simulink model "RobustFormationControl_IntegerModel_under_Dis"  (R2023a)
settings: Solver=ode3  StartTime=0.0  StopTime=30  FixedStep=0.0001  RelTol=1e-3
InitFcn:
  | % % Parameters for the fractional order NTFSMC:
  | % Sliding Surface " Sx, Sy, and Sz ":
  | %------------------------
  | % 10
  | % 10
  | cx = 2*[4 4 4];
  | cxx = 1*[0.01 0.01 0.01];
  | 
  | cx1 = cx(1);
  | cy1 = cx(2);
  | cz1 = cx(3);
  | 
  | cx2 = cxx(1);
  | cy2 = cxx(2);
  | cz2 = cxx(3);
  | 
  | alpha1 = [0.6 0.6 0.6];
  | alpha2 = [0.1 0.1 0.1];
  | 
  | gammaX = [3 3 3];
  | gx  = gammaX(1);
  | gy = gammaX(2);
  | gz = gammaX(3);
  | 
  | p = 10;
  | q = 10;
  | 
  | % Sliding Surface " S_Phi , S_Theta, and  S_Psi":
  | %------------------------
  | cP = 2*[4 4 4];
  | cPP = 1*[0.01 0.01 0.01 0.01];
  | 
  | cPhi1 = cP(1);
  | cTheta1 = cP(2);
  | cPsi1 = cP(3);
  | 
  | cPhi2 = cPP(1);
  | cTheta2 = cPP(2);
  | cPsi2 = cPP(3);
  | gammaP = [3 3 3];
  | 
  | %=========================
  | %=========================
  | SigmaX = 1*[0.01 0.01 0.01];
  | SigmaXX =1*[1 1 1];
  | 
  | Sigma1X = SigmaX(1);
  | Sigma1Y = SigmaX(2);
  | Sigma1Z = SigmaX(3);
  | %-----
  | Sigma2X = SigmaXX(1);
  | Sigma2Y = SigmaXX(2);
  | Sigma2Z = SigmaXX(3);
  | 
  | 
  | SigmaP = 1*[0.01 0.01 0.01];
  | SigmaPP =1*[1 1 1];
  | 
  | Sigma1Phi   = SigmaP(1);
  | Sigma1Theta = SigmaP(2);
  | ... (+80 lines)
values from neighbouring files (symbols this model uses):
  a1 = (Iyy - Izz)/Ixx    (= -0.812397034596)    [init_quadrotor_params.m]
  a2 = (Izz - Ixx)/Iyy    (= 0.812397034596)    [init_quadrotor_params.m]
  a3 = (Ixx - Iyy)/Izz    (= 0)    [init_quadrotor_params.m]
  a4 = - Ktx/m    (= -0.00114547325103)    [init_quadrotor_params.m]
  a5 = - Kty/m    (= -0.00114547325103)    [init_quadrotor_params.m]
  a6 = - Ktz/m    (= -0.00130740740741)    [init_quadrotor_params.m]
  b = 2.980e-5    (= 2.98e-05)    [init_quadrotor_params.m]
  b1 = - Jr/Ixx    (= -0.00584534596376)    [init_quadrotor_params.m]
  b2 = Jr/Iyy    (= 0.00584534596376)    [init_quadrotor_params.m]
  b3 = - Kfz/Izz    (= -0.0721963413248)    [init_quadrotor_params.m]
  b4 = 1/m    (= 2.05761316872)    [init_quadrotor_params.m]
  b5 = 1/m    (= 2.05761316872)    [init_quadrotor_params.m]
  b6 = 1/m    (= 2.05761316872)    [init_quadrotor_params.m]
  c1 = - Kfx/Ixx    (= -0.114641680395)    [init_quadrotor_params.m]
  c2 = - Kfy/Iyy    (= -0.114641680395)    [init_quadrotor_params.m]
  c3 = 1/Izz    (= 113.62345188)    [init_quadrotor_params.m]
  d = 1.12e-06    [init_quadrotor_params.m]
  d1 = L/Ixx    (= 46.334431631)    [init_quadrotor_params.m]
  d2 = L/Iyy    (= 46.334431631)    [init_quadrotor_params.m]
  g = 9.81    [init_quadrotor_params.m]
  Ixx = 4.856e-3    (= 0.004856)    [init_quadrotor_params.m]
  Iyy = 4.856e-3    (= 0.004856)    [init_quadrotor_params.m]
  Izz = 8.801e-3    (= 0.008801)    [init_quadrotor_params.m]
  Jr = 2.8385e-5    (= 2.8385e-05)    [init_quadrotor_params.m]
  Kfx = 5.567e-4    (= 0.0005567)    [init_quadrotor_params.m]
  Kfy = 5.567e-4    (= 0.0005567)    [init_quadrotor_params.m]
  Kfz = 6.354e-4    (= 0.0006354)    [init_quadrotor_params.m]
  Ktx = 5.5670e-4    (= 0.0005567)    [init_quadrotor_params.m]
  Kty = 5.5670e-4    (= 0.0005567)    [init_quadrotor_params.m]
  Ktz = 6.3540e-4    (= 0.0006354)    [init_quadrotor_params.m]
  L = 0.225    [init_quadrotor_params.m]
  m = 0.486    [init_quadrotor_params.m]
libraries: fod x120, eeStairGenerator x5
(part 3 of 9)

== system RobustFormationControl_IntegerModel_under_Dis/Integer Leader and four followers/Follower 3 System/Follower 2 Quadrotor Model/Quadrotor Dynamic System ==
  U1 : Inport
  U2 : Inport  Port=2
  U3 : Inport  Port=3
  U4 : Inport  Port=4
  Ux : Inport  Port=5
  Uy : Inport  Port=6
  Omega : Inport  Port=7
  Rotational System : Subsystem
  Translational System : Subsystem
  x = x7 : Outport  VectorParamsAs1DForOutWhenUnconnected=off
  y = x9 : Outport  Port=2  VectorParamsAs1DForOutWhenUnconnected=off
  z = x11 : Outport  Port=3  VectorParamsAs1DForOutWhenUnconnected=off
  Phi : Outport  Port=4  VectorParamsAs1DForOutWhenUnconnected=off
  Theta : Outport  Port=5  VectorParamsAs1DForOutWhenUnconnected=off
  Psi : Outport  Port=6  VectorParamsAs1DForOutWhenUnconnected=off
  x2 : Outport  Port=7  VectorParamsAs1DForOutWhenUnconnected=off
  x4 : Outport  Port=8  VectorParamsAs1DForOutWhenUnconnected=off
  x6 : Outport  Port=9  VectorParamsAs1DForOutWhenUnconnected=off
  xdot = x8 : Outport  Port=10  VectorParamsAs1DForOutWhenUnconnected=off
  ydot = x10 : Outport  Port=11  VectorParamsAs1DForOutWhenUnconnected=off
  zdot = x12 : Outport  Port=12  VectorParamsAs1DForOutWhenUnconnected=off
  wires:
  Rotational System/6(x6) -> x6/1
  Rotational System/5(x4) -> x4/1
  Rotational System/4(x2) -> x2/1
  Translational System/6(zdot or x12) -> zdot = x12/1
  Translational System/5(ydot or x10) -> ydot = x10/1
  Translational System/4(xdot or x8) -> xdot = x8/1
  Uy/1 -> Translational System/3(Uy)
  Ux/1 -> Translational System/2(Ux)
  Translational System/1(x or x7) -> x = x7/1  "X"
  Translational System/2(y or x9) -> y = x9/1  "Y"
  U1/1 -> Translational System/1(U1)
  Omega/1 -> Rotational System/4(Omega)
  Translational System/3(z or x11) -> z = x11/1  "Z"
  Rotational System/3(Psi or x5) -> Psi/1  "Psi"
  U3/1 -> Rotational System/2(U3)
  U2/1 -> Rotational System/1(U2)
  U4/1 -> Rotational System/3(U4)
  Rotational System/1(Phi or x1) -> Phi/1, Translational System/4(x1)  "Phi"
  Rotational System/2(Theta or x3) -> Theta/1, Translational System/5(x3)  "Theta"

== system RobustFormationControl_IntegerModel_under_Dis/Integer Leader and four followers/Follower 4 System/Desired Values/Helical Trajectry ==
  t : Inport
  Gain2 : Gain  Gain=0.2
  Step1 : Step  Time=0  SampleTime=0
  Trigonometric Function : Trigonometry
  Trigonometric Function1 : Trigonometry  Operator=cos
  xd : Outport  VectorParamsAs1DForOutWhenUnconnected=off
  yd : Outport  Port=2  VectorParamsAs1DForOutWhenUnconnected=off
  zd : Outport  Port=3  VectorParamsAs1DForOutWhenUnconnected=off
  Psi_d : Outport  Port=4  VectorParamsAs1DForOutWhenUnconnected=off
  wires:
  t/1 -> Trigonometric Function1/1, Trigonometric Function/1, Gain2/1
  Gain2/1 -> zd/1
  Step1/1 -> Psi_d/1
  Trigonometric Function1/1 -> xd/1
  Trigonometric Function/1 -> yd/1

== system RobustFormationControl_IntegerModel_under_Dis/Integer Leader and four followers/Follower 4 System/Desired Values/Helical Trajectry1 ==
  t : Inport
  Gain : Gain  Gain=dis
  Gain1 : Gain  Gain=2*pi/15
  Gain2 : Gain  Gain=1/15
  Gain3 : Gain  Gain=2*pi/15
  Scope : Scope
  Step : Step  Time=0  After=0  SampleTime=0.03
  Step1 : Step  Time=0  SampleTime=0
  Step2 : Step  Time=5  After=0.5  SampleTime=0.03
  Step3 : Step  Time=10  After=0.5  SampleTime=0.03
  Sum : Sum  Inputs=++-
  Sum1 : Sum  Inputs=|++
  Trigonometric Function : Trigonometry  Operator=cos
  Trigonometric Function1 : Trigonometry
  xd : Outport  VectorParamsAs1DForOutWhenUnconnected=off
  yd : Outport  Port=2  VectorParamsAs1DForOutWhenUnconnected=off
  zd : Outport  Port=3  VectorParamsAs1DForOutWhenUnconnected=off
  Psi_d : Outport  Port=4  VectorParamsAs1DForOutWhenUnconnected=off
  wires:
  t/1 -> Gain1/1, Gain3/1, Gain2/1
  Gain2/1 -> zd/1
  Step1/1 -> Psi_d/1
  Trigonometric Function1/1 -> yd/1
  Step/1 -> Sum/1
  Sum/1 -> Gain/1, Scope/1
  Step2/1 -> Sum/2
  Step3/1 -> Sum/3
  Sum1/1 -> xd/1
  Trigonometric Function/1 -> Sum1/2
  Gain/1 -> Sum1/1
  Gain1/1 -> Trigonometric Function/1
  Gain3/1 -> Trigonometric Function1/1

== system RobustFormationControl_IntegerModel_under_Dis/Integer Leader and four followers/Follower 4 System/Desired Values/Step Inputs Trajectry ==
  Step : Step  Time=0  After=3  SampleTime=0
  Step1 : Step  Time=0  After=5  SampleTime=0
  Step2 : Step  Time=0  SampleTime=0
  Step3 : Step  Time=0  After=2  SampleTime=0
  xd : Outport  VectorParamsAs1DForOutWhenUnconnected=off
  yd : Outport  Port=2  VectorParamsAs1DForOutWhenUnconnected=off
  zd : Outport  Port=3  VectorParamsAs1DForOutWhenUnconnected=off
  Psi_d : Outport  Port=4  VectorParamsAs1DForOutWhenUnconnected=off
  wires:
  Step2/1 -> xd/1
  Step3/1 -> yd/1
  Step/1 -> zd/1
  Step1/1 -> Psi_d/1

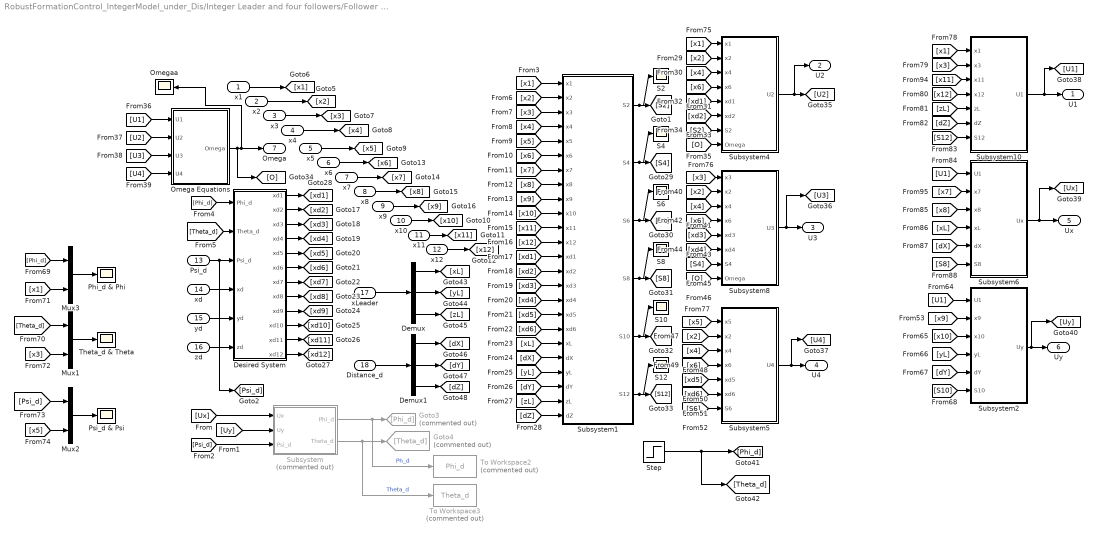
== system RobustFormationControl_IntegerModel_under_Dis/Integer Leader and four followers/Follower 4 System/Follower 2 Quadrotor Model/Control Module1 ==
  x1 : Inport
  x2 : Inport  Port=2
  x3 : Inport  Port=3
  x4 : Inport  Port=4
  x5 : Inport  Port=5
  x6 : Inport  Port=6
  x7 : Inport  Port=7
  x8 : Inport  Port=8
  x9 : Inport  Port=9
  x10 : Inport  Port=10
  x11 : Inport  Port=11
  x12 : Inport  Port=12
  Psi_d : Inport  Port=13
  " xd" : Inport  Port=14
  yd : Inport  Port=15
  " zd" : Inport  Port=16
  xLeader : Inport  Port=17
  Distance_d : Inport  Port=18
  " Phi_d & Phi" : Scope
  " Theta_d & Theta" : Scope
  Demux : Demux  Outputs=3
  Demux1 : Demux  Outputs=3
  Desired System : Subsystem
  Goto3 : Goto  Commented=on  GotoTag=Phi_d
  Goto4 : Goto  Commented=on  GotoTag=Theta_d
  Mux1 : Mux  Inputs=2
  Mux2 : Mux  Inputs=2
  Mux3 : Mux  Inputs=2
  Omega Equations : Subsystem
  Omegaa : Scope
  Psi_d & Psi : Scope
  S{4,6,8,10,12} (5 alike) : Scope
  "S2 " : Scope
  Step : Step  Time=0  After=0.001  SampleTime=0
  Subsystem : Subsystem  Commented=on
  Subsystem1 : Subsystem
  Subsystem10 : Subsystem
  Subsystem2 : Subsystem
  Subsystem4 : Subsystem
  Subsystem5 : Subsystem
  Subsystem6 : Subsystem
  Subsystem8 : Subsystem
  To Workspace2 : ToWorkspace  Commented=on  VariableName=Phi_d  SampleTime=-1
  To Workspace3 : ToWorkspace  Commented=on  VariableName=Theta_d  SampleTime=-1
  U1 : Outport  VectorParamsAs1DForOutWhenUnconnected=off
  U2 : Outport  Port=2  VectorParamsAs1DForOutWhenUnconnected=off
  U3 : Outport  Port=3  VectorParamsAs1DForOutWhenUnconnected=off
  U4 : Outport  Port=4  VectorParamsAs1DForOutWhenUnconnected=off
  Ux : Outport  Port=5  VectorParamsAs1DForOutWhenUnconnected=off
  Uy : Outport  Port=6  VectorParamsAs1DForOutWhenUnconnected=off
  Omega : Outport  Port=7  VectorParamsAs1DForOutWhenUnconnected=off
  wires:
  Omega Equations/1(Omega) -> [O], Omegaa/1, Omega/1
  [Ux] -> Subsystem/1(Ux)
  [Uy] -> Subsystem/2(Uy)
  [Psi_d] -> Subsystem/3(Psi_d)
  Subsystem/1(Phi_d) -> To Workspace2/1, Goto3/1  "Ph_d"
  Subsystem/2(Theta_d) -> To Workspace3/1, Goto4/1  "Theta_d"
  [xd1] -> Subsystem1/13(xd1)
  [xd2] -> Subsystem1/14(xd2)
  [xd3] -> Subsystem1/15(xd3)
  [xd4] -> Subsystem1/16(xd4)
  [xd5] -> Subsystem1/17(xd5)
  [xd6] -> Subsystem1/18(xd6)
  [xL] -> Subsystem1/19(xL)
  [dX] -> Subsystem1/20(dX)
  [yL] -> Subsystem1/21(yL)
  [dY] -> Subsystem1/22(dY)
  [zL] -> Subsystem1/23(zL)
  [dZ] -> Subsystem1/24(dZ)
  x9/1 -> [x9]
  x5/1 -> [x5]
  x6/1 -> [x6]
  x1/1 -> [x1]
  x4/1 -> [x4]
  x3/1 -> [x3]
  x11/1 -> [x11]
  x10/1 -> [x10]
  x8/1 -> [x8]
  x2/1 -> [x2]
  x7/1 -> [x7]
  x12/1 -> [x12]
  [Phi_d] -> Desired System/1(Phi_d)
  [Theta_d] -> Desired System/2(Theta_d)
  Psi_d/1 -> [Psi_d], Desired System/3(Psi_d)
  " xd"/1 -> Desired System/4(xd)
  yd/1 -> Desired System/5(yd)
  Desired System/2(xd2) -> [xd2]
  Desired System/3(xd3) -> [xd3]
  Desired System/4(xd4) -> [xd4]
  Desired System/5(xd5) -> [xd5]
  Desired System/6(xd6) -> [xd6]
  Desired System/7(xd7) -> [xd7]
  Desired System/8(xd8) -> [xd8]
  Desired System/9(xd9) -> [xd9]
  Desired System/10(xd10) -> [xd10]
  Desired System/11(xd11) -> [xd11]
  Desired System/12(xd12) -> [xd12]
  Desired System/1(xd1) -> [xd1]
  " zd"/1 -> Desired System/6(zd)
  [x1] -> Subsystem1/1(x1)
  [x12] -> Subsystem1/12(x12)
  [x11] -> Subsystem1/11(x11)
  [x10] -> Subsystem1/10(x10)
  [x9] -> Subsystem1/9(x9)
  [x8] -> Subsystem1/8(x8)
  [x7] -> Subsystem1/7(x7)
  [x6] -> Subsystem1/6(x6)
  [x5] -> Subsystem1/5(x5)
  [x4] -> Subsystem1/4(x4)
  [x3] -> Subsystem1/3(x3)
  [x2] -> Subsystem1/2(x2)
  Subsystem1/1(S2) -> "S2 "/1, [S2]
  Subsystem1/2(S4) -> S4/1, [S4]
  Subsystem1/3(S6) -> S6/1, [S6]
  Subsystem1/4(S8) -> S8/1, [S8]
  Subsystem1/5(S10) -> S10/1, [S10]
  Subsystem1/6(S12) -> S12/1, [S12]
  [U1] -> Omega Equations/1(U1)
  [U4] -> Omega Equations/4(U4)
  [U3] -> Omega Equations/3(U3)
  [U2] -> Omega Equations/2(U2)
  Step/1 -> [Theta_d], [Phi_d]
  Mux3/1 -> " Phi_d & Phi"/1
  Mux1/1 -> " Theta_d & Theta"/1
  [Phi_d] -> Mux3/1
  [Theta_d] -> Mux1/1
  [x1] -> Mux3/2
  [x3] -> Mux1/2
  Mux2/1 -> Psi_d & Psi/1
  [Psi_d] -> Mux2/1
  [x5] -> Mux2/2
  Demux/1 -> [xL]
  Demux/2 -> [yL]
  Demux/3 -> [zL]
  Demux1/2 -> [dY]
  Demux1/3 -> [dZ]
  Demux1/1 -> [dX]
  xLeader/1 -> Demux/1
  Distance_d/1 -> Demux1/1
  [x2] -> Subsystem4/2(x2)
  [O] -> Subsystem4/8(Omega)
  [x6] -> Subsystem4/4(x6)
  [xd4] -> Subsystem8/6(xd4)
  [xd2] -> Subsystem4/6(xd2)
  [x3] -> Subsystem8/1(x3)
  Subsystem8/1(U3) -> [U3], U3/1
  Subsystem4/1(U2) -> U2/1, [U2]
  [x1] -> Subsystem4/1(x1)
  [x5] -> Subsystem5/1(x5)
  [O] -> Subsystem8/8(Omega)
  [x6] -> Subsystem5/4(x6)
  [S2] -> Subsystem4/7(S2)
  [xd3] -> Subsystem8/5(xd3)
  [S6] -> Subsystem5/7(S6)
  [xd1] -> Subsystem4/5(xd1)
  Subsystem5/1(U4) -> [U4], U4/1
  [x2] -> Subsystem5/2(x2)
  [x6] -> Subsystem8/4(x6)
  [xd6] -> Subsystem5/6(xd6)
  [x2] -> Subsystem8/2(x2)
  [S4] -> Subsystem8/7(S4)
  [x4] -> Subsystem8/3(x4)
  [xd5] -> Subsystem5/5(xd5)
  [x4] -> Subsystem4/3(x4)
  [x4] -> Subsystem5/3(x4)
  Subsystem10/1(U1) -> [U1], U1/1
  [x12] -> Subsystem10/4(x12)
  [x11] -> Subsystem10/3(x11)
  [dZ] -> Subsystem10/6(dZ)
  [S12] -> Subsystem10/7(S12)
  Subsystem6/1(Ux) -> [Ux], Ux/1
  [x1] -> Subsystem10/1(x1)
  [dX] -> Subsystem6/5(dX)
  [zL] -> Subsystem10/5(zL)
  [S8] -> Subsystem6/6(S8)
  [xL] -> Subsystem6/4(xL)
  [x8] -> Subsystem6/3(x8)
  [x7] -> Subsystem6/2(x7)
  [x3] -> Subsystem10/2(x3)
  [U1] -> Subsystem6/1(U1)
  Subsystem2/1(Uy) -> [Uy], Uy/1
  [U1] -> Subsystem2/1(U1)
  [x10] -> Subsystem2/3(x10)
  [yL] -> Subsystem2/4(yL)
  [S10] -> Subsystem2/6(S10)
  [dY] -> Subsystem2/5(dY)
  [x9] -> Subsystem2/2(x9)

== system RobustFormationControl_IntegerModel_under_Dis/Integer Leader and four followers/Follower 4 System/Follower 2 Quadrotor Model/Quadrotor Dynamic System ==
  U1 : Inport
  U2 : Inport  Port=2
  U3 : Inport  Port=3
  U4 : Inport  Port=4
  Ux : Inport  Port=5
  Uy : Inport  Port=6
  Omega : Inport  Port=7
  Rotational System : Subsystem
  Translational System : Subsystem
  x = x7 : Outport  VectorParamsAs1DForOutWhenUnconnected=off
  y = x9 : Outport  Port=2  VectorParamsAs1DForOutWhenUnconnected=off
  z = x11 : Outport  Port=3  VectorParamsAs1DForOutWhenUnconnected=off
  Phi : Outport  Port=4  VectorParamsAs1DForOutWhenUnconnected=off
  Theta : Outport  Port=5  VectorParamsAs1DForOutWhenUnconnected=off
  Psi : Outport  Port=6  VectorParamsAs1DForOutWhenUnconnected=off
  x2 : Outport  Port=7  VectorParamsAs1DForOutWhenUnconnected=off
  x4 : Outport  Port=8  VectorParamsAs1DForOutWhenUnconnected=off
  x6 : Outport  Port=9  VectorParamsAs1DForOutWhenUnconnected=off
  xdot = x8 : Outport  Port=10  VectorParamsAs1DForOutWhenUnconnected=off
  ydot = x10 : Outport  Port=11  VectorParamsAs1DForOutWhenUnconnected=off
  zdot = x12 : Outport  Port=12  VectorParamsAs1DForOutWhenUnconnected=off
  wires:
  Rotational System/2(Theta or x3) -> Translational System/5(x3), Theta/1  "Theta"
  Rotational System/1(Phi or x1) -> Translational System/4(x1), Phi/1  "Phi"
  U4/1 -> Rotational System/3(U4)
  U2/1 -> Rotational System/1(U2)
  U3/1 -> Rotational System/2(U3)
  Rotational System/3(Psi or x5) -> Psi/1  "Psi"
  Translational System/3(z or x11) -> z = x11/1  "Z"
  Omega/1 -> Rotational System/4(Omega)
  U1/1 -> Translational System/1(U1)
  Translational System/2(y or x9) -> y = x9/1  "Y"
  Translational System/1(x or x7) -> x = x7/1  "X"
  Ux/1 -> Translational System/2(Ux)
  Uy/1 -> Translational System/3(Uy)
  Translational System/4(xdot or x8) -> xdot = x8/1
  Translational System/5(ydot or x10) -> ydot = x10/1
  Translational System/6(zdot or x12) -> zdot = x12/1
  Rotational System/4(x2) -> x2/1
  Rotational System/5(x4) -> x4/1
  Rotational System/6(x6) -> x6/1

== system RobustFormationControl_IntegerModel_under_Dis/Integer Leader and four followers/Leader System/Desired Values/Circular Trajectry ==
  t : Inport
  Gain1 : Gain
  Step : Step  Time=0  SampleTime=0
  Step1 : Step  Time=0  SampleTime=0
  Trigonometric Function : Trigonometry  Operator=cos
  Trigonometric Function1 : Trigonometry
  xd : Outport  VectorParamsAs1DForOutWhenUnconnected=off
  yd : Outport  Port=2  VectorParamsAs1DForOutWhenUnconnected=off
  zd : Outport  Port=3  VectorParamsAs1DForOutWhenUnconnected=off
  Psi_d : Outport  Port=4  VectorParamsAs1DForOutWhenUnconnected=off
  wires:
  t/1 -> Gain1/1
  Gain1/1 -> Trigonometric Function1/1, Trigonometric Function/1
  Trigonometric Function/1 -> xd/1
  Trigonometric Function1/1 -> yd/1
  Step/1 -> zd/1
  Step1/1 -> Psi_d/1

== system RobustFormationControl_IntegerModel_under_Dis/Integer Leader and four followers/Leader System/Desired Values/Helical Trajectry ==
  t : Inport
  Constant : Constant  Value=0
  Gain : Gain  Gain=dis
  Gain1 : Gain  Gain=2*pi/15
  Gain2 : Gain  Gain=1/15
  Gain3 : Gain  Gain=2*pi/15
  Scope : Scope
  Step : Step  Time=0  After=0  SampleTime=0.03
  Step1 : Step  Time=0  SampleTime=0
  Step2 : Step  Time=5  After=0.5  SampleTime=0.03
  Step3 : Step  Time=10  After=0.5  SampleTime=0.03
  Sum : Sum  Inputs=++-
  Sum1 : Sum  Inputs=|+++
  Trigonometric Function : Trigonometry  Operator=cos
  Trigonometric Function1 : Trigonometry
  xd : Outport  VectorParamsAs1DForOutWhenUnconnected=off
  yd : Outport  Port=2  VectorParamsAs1DForOutWhenUnconnected=off
  zd : Outport  Port=3  VectorParamsAs1DForOutWhenUnconnected=off
  Psi_d : Outport  Port=4  VectorParamsAs1DForOutWhenUnconnected=off
  wires:
  t/1 -> Gain1/1, Gain3/1, Gain2/1
  Gain2/1 -> zd/1
  Step1/1 -> Psi_d/1
  Trigonometric Function1/1 -> yd/1
  Step/1 -> Sum/1
  Sum/1 -> Gain/1, Scope/1
  Step2/1 -> Sum/2
  Step3/1 -> Sum/3
  Sum1/1 -> xd/1
  Trigonometric Function/1 -> Sum1/2
  Gain/1 -> Sum1/1
  Gain1/1 -> Trigonometric Function/1
  Gain3/1 -> Trigonometric Function1/1
  Constant/1 -> Sum1/3

== system RobustFormationControl_IntegerModel_under_Dis/Integer Leader and four followers/Leader System/Desired Values/Step Inputs Trajectry ==
  Step : Step  Time=0  After=3  SampleTime=0
  Step1 : Step  Time=0  After=5  SampleTime=0
  Step2 : Step  Time=0  SampleTime=0
  Step3 : Step  Time=0  After=2  SampleTime=0
  xd : Outport  VectorParamsAs1DForOutWhenUnconnected=off
  yd : Outport  Port=2  VectorParamsAs1DForOutWhenUnconnected=off
  zd : Outport  Port=3  VectorParamsAs1DForOutWhenUnconnected=off
  Psi_d : Outport  Port=4  VectorParamsAs1DForOutWhenUnconnected=off
  wires:
  Step2/1 -> xd/1
  Step3/1 -> yd/1
  Step/1 -> zd/1
  Step1/1 -> Psi_d/1

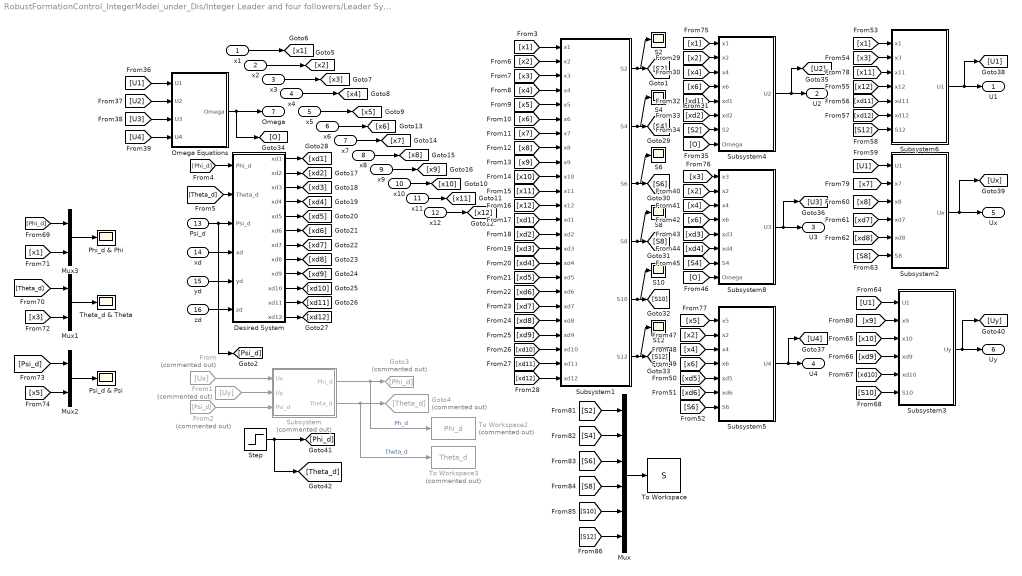
== system RobustFormationControl_IntegerModel_under_Dis/Integer Leader and four followers/Leader System/Integer Model/Control Module1 ==
  x1 : Inport
  x2 : Inport  Port=2
  x3 : Inport  Port=3
  x4 : Inport  Port=4
  x5 : Inport  Port=5
  x6 : Inport  Port=6
  x7 : Inport  Port=7
  x8 : Inport  Port=8
  x9 : Inport  Port=9
  x10 : Inport  Port=10
  x11 : Inport  Port=11
  x12 : Inport  Port=12
  Psi_d : Inport  Port=13
  " xd" : Inport  Port=14
  yd : Inport  Port=15
  " zd" : Inport  Port=16
  " Phi_d & Phi" : Scope
  " Theta_d & Theta" : Scope
  Desired System : Subsystem
  From : From  Commented=on  GotoTag=Ux
  From1 : From  Commented=on  GotoTag=Uy
  From2 : From  Commented=on  GotoTag=Psi_d
  Goto3 : Goto  Commented=on  GotoTag=Phi_d
  Goto4 : Goto  Commented=on  GotoTag=Theta_d
  Mux : Mux  Inputs=6
  Mux1 : Mux  Inputs=2
  Mux2 : Mux  Inputs=2
  Mux3 : Mux  Inputs=2
  Omega Equations : Subsystem
  Psi_d & Psi : Scope
  S{4,6,8,10,12} (5 alike) : Scope
  "S2 " : Scope
  Step : Step  Time=0  After=0.001  SampleTime=0
  Subsystem : Subsystem  Commented=on
  Subsystem1 : Subsystem
  Subsystem2 : Subsystem
  Subsystem3 : Subsystem
  Subsystem4 : Subsystem
  Subsystem5 : Subsystem
  Subsystem6 : Subsystem
  Subsystem8 : Subsystem
  To Workspace : ToWorkspace  VariableName=S  SampleTime=-1
  To Workspace2 : ToWorkspace  Commented=on  VariableName=Phi_d  SampleTime=-1
  To Workspace3 : ToWorkspace  Commented=on  VariableName=Theta_d  SampleTime=-1
  U1 : Outport  VectorParamsAs1DForOutWhenUnconnected=off
  U2 : Outport  Port=2  VectorParamsAs1DForOutWhenUnconnected=off
  U3 : Outport  Port=3  VectorParamsAs1DForOutWhenUnconnected=off
  U4 : Outport  Port=4  VectorParamsAs1DForOutWhenUnconnected=off
  Ux : Outport  Port=5  VectorParamsAs1DForOutWhenUnconnected=off
  Uy : Outport  Port=6  VectorParamsAs1DForOutWhenUnconnected=off
  Omega : Outport  Port=7  VectorParamsAs1DForOutWhenUnconnected=off
  wires:
  Omega Equations/1(Omega) -> [O], Omega/1
  From/1 -> Subsystem/1(Ux)
  From1/1 -> Subsystem/2(Uy)
  From2/1 -> Subsystem/3(Psi_d)
  Subsystem/1(Phi_d) -> To Workspace2/1, Goto3/1  "Ph_d"
  Subsystem/2(Theta_d) -> To Workspace3/1, Goto4/1  "Theta_d"
  [xd1] -> Subsystem1/13(xd1)
  [xd2] -> Subsystem1/14(xd2)
  [xd3] -> Subsystem1/15(xd3)
  [xd4] -> Subsystem1/16(xd4)
  [xd5] -> Subsystem1/17(xd5)
  [xd6] -> Subsystem1/18(xd6)
  [xd7] -> Subsystem1/19(xd7)
  [xd8] -> Subsystem1/20(xd8)
  [xd9] -> Subsystem1/21(xd9)
  [xd10] -> Subsystem1/22(xd10)
  [xd11] -> Subsystem1/23(xd11)
  [xd12] -> Subsystem1/24(xd12)
  x9/1 -> [x9]
  x5/1 -> [x5]
  x6/1 -> [x6]
  x1/1 -> [x1]
  x4/1 -> [x4]
  x3/1 -> [x3]
  x11/1 -> [x11]
  x10/1 -> [x10]
  x8/1 -> [x8]
  x2/1 -> [x2]
  x7/1 -> [x7]
  x12/1 -> [x12]
  [Phi_d] -> Desired System/1(Phi_d)
  [Theta_d] -> Desired System/2(Theta_d)
  Psi_d/1 -> [Psi_d], Desired System/3(Psi_d)
  " xd"/1 -> Desired System/4(xd)
  yd/1 -> Desired System/5(yd)
  Desired System/2(xd2) -> [xd2]
  Desired System/3(xd3) -> [xd3]
  Desired System/4(xd4) -> [xd4]
  Desired System/5(xd5) -> [xd5]
  Desired System/6(xd6) -> [xd6]
  Desired System/7(xd7) -> [xd7]
  Desired System/8(xd8) -> [xd8]
  Desired System/9(xd9) -> [xd9]
  Desired System/10(xd10) -> [xd10]
  Desired System/11(xd11) -> [xd11]
  Desired System/12(xd12) -> [xd12]
  Desired System/1(xd1) -> [xd1]
  " zd"/1 -> Desired System/6(zd)
  [x1] -> Subsystem1/1(x1)
  [x12] -> Subsystem1/12(x12)
  [x11] -> Subsystem1/11(x11)
  [x10] -> Subsystem1/10(x10)
  [x9] -> Subsystem1/9(x9)
  [x8] -> Subsystem1/8(x8)
  [x7] -> Subsystem1/7(x7)
  [x6] -> Subsystem1/6(x6)
  [x5] -> Subsystem1/5(x5)
  [x4] -> Subsystem1/4(x4)
  [x3] -> Subsystem1/3(x3)
  [x2] -> Subsystem1/2(x2)
  Subsystem6/1(U1) -> [U1], U1/1
  Subsystem4/1(U2) -> [U2], U2/1
  Subsystem2/1(Ux) -> [Ux], Ux/1
  Subsystem3/1(Uy) -> Uy/1, [Uy]
  Subsystem1/1(S2) -> "S2 "/1, [S2]
  Subsystem1/2(S4) -> S4/1, [S4]
  Subsystem1/3(S6) -> S6/1, [S6]
  Subsystem1/4(S8) -> S8/1, [S8]
  Subsystem1/5(S10) -> S10/1, [S10]
  Subsystem1/6(S12) -> S12/1, [S12]
  [x2] -> Subsystem4/2(x2)
  [x4] -> Subsystem4/3(x4)
  [x6] -> Subsystem4/4(x6)
  [xd1] -> Subsystem4/5(xd1)
  [xd2] -> Subsystem4/6(xd2)
  [S2] -> Subsystem4/7(S2)
  [O] -> Subsystem4/8(Omega)
  Subsystem5/1(U4) -> [U4], U4/1
  [U1] -> Omega Equations/1(U1)
  [U4] -> Omega Equations/4(U4)
  [U3] -> Omega Equations/3(U3)
  [U2] -> Omega Equations/2(U2)
  [xd4] -> Subsystem8/6(xd4)
  [S4] -> Subsystem8/7(S4)
  [x6] -> Subsystem8/4(x6)
  [x2] -> Subsystem8/2(x2)
  [xd3] -> Subsystem8/5(xd3)
  [x4] -> Subsystem8/3(x4)
  [O] -> Subsystem8/8(Omega)
  [x6] -> Subsystem5/4(x6)
  [x2] -> Subsystem5/2(x2)
  [x4] -> Subsystem5/3(x4)
  [S6] -> Subsystem5/7(S6)
  [xd6] -> Subsystem5/6(xd6)
  [xd5] -> Subsystem5/5(xd5)
  Step/1 -> [Theta_d], [Phi_d]
  Mux3/1 -> " Phi_d & Phi"/1
  Mux1/1 -> " Theta_d & Theta"/1
  [Phi_d] -> Mux3/1
  [Theta_d] -> Mux1/1
  [x1] -> Mux3/2
  [x3] -> Mux1/2
  Mux2/1 -> Psi_d & Psi/1
  [Psi_d] -> Mux2/1
  [x5] -> Mux2/2
  [x1] -> Subsystem4/1(x1)
  [x3] -> Subsystem8/1(x3)
  Subsystem8/1(U3) -> [U3], U3/1
  [x5] -> Subsystem5/1(x5)
  [x1] -> Subsystem6/1(x1)
  [x3] -> Subsystem6/2(x3)
  [x12] -> Subsystem6/4(x12)
  [xd11] -> Subsystem6/5(xd11)
  [xd12] -> Subsystem6/6(xd12)
  [S12] -> Subsystem6/7(S12)
  [x11] -> Subsystem6/3(x11)
  [U1] -> Subsystem2/1(U1)
  [x7] -> Subsystem2/2(x7)
  [x8] -> Subsystem2/3(x8)
  [xd7] -> Subsystem2/4(xd7)
  [xd8] -> Subsystem2/5(xd8)
  [S8] -> Subsystem2/6(S8)
  [U1] -> Subsystem3/1(U1)
  [x10] -> Subsystem3/3(x10)
  [xd9] -> Subsystem3/4(xd9)
  [xd10] -> Subsystem3/5(xd10)
  [S10] -> Subsystem3/6(S10)
  [x9] -> Subsystem3/2(x9)
  [S2] -> Mux/1
  [S4] -> Mux/2
  [S6] -> Mux/3
  [S8] -> Mux/4
  [S10] -> Mux/5
  [S12] -> Mux/6
  Mux/1 -> To Workspace/1

== system RobustFormationControl_IntegerModel_under_Dis/Integer Leader and four followers/Leader System/Integer Model/Quadrotor Dynamic System ==
  U1 : Inport
  U2 : Inport  Port=2
  U3 : Inport  Port=3
  U4 : Inport  Port=4
  Ux : Inport  Port=5
  Uy : Inport  Port=6
  Omega : Inport  Port=7
  Rotational System : Subsystem
  Translational System : Subsystem
  x = x7 : Outport  VectorParamsAs1DForOutWhenUnconnected=off
  y = x9 : Outport  Port=2  VectorParamsAs1DForOutWhenUnconnected=off
  z = x11 : Outport  Port=3  VectorParamsAs1DForOutWhenUnconnected=off
  Phi : Outport  Port=4  VectorParamsAs1DForOutWhenUnconnected=off
  Theta : Outport  Port=5  VectorParamsAs1DForOutWhenUnconnected=off
  Psi : Outport  Port=6  VectorParamsAs1DForOutWhenUnconnected=off
  x2 : Outport  Port=7  VectorParamsAs1DForOutWhenUnconnected=off
  x4 : Outport  Port=8  VectorParamsAs1DForOutWhenUnconnected=off
  x6 : Outport  Port=9  VectorParamsAs1DForOutWhenUnconnected=off
  xdot = x8 : Outport  Port=10  VectorParamsAs1DForOutWhenUnconnected=off
  ydot = x10 : Outport  Port=11  VectorParamsAs1DForOutWhenUnconnected=off
  zdot = x12 : Outport  Port=12  VectorParamsAs1DForOutWhenUnconnected=off
  wires:
  Rotational System/2(Theta or x3) -> Translational System/5(x3), Theta/1  "Theta"
  Rotational System/1(Phi or x1) -> Translational System/4(x1), Phi/1  "Phi"
  U4/1 -> Rotational System/3(U4)
  U2/1 -> Rotational System/1(U2)
  U3/1 -> Rotational System/2(U3)
  Rotational System/3(Psi or x5) -> Psi/1  "Psi"
  Translational System/3(z or x11) -> z = x11/1  "Z"
  Omega/1 -> Rotational System/4(Omega)
  U1/1 -> Translational System/1(U1)
  Translational System/2(y or x9) -> y = x9/1  "Y"
  Translational System/1(x or x7) -> x = x7/1  "X"
  Ux/1 -> Translational System/2(Ux)
  Uy/1 -> Translational System/3(Uy)
  Translational System/4(xdot or x8) -> xdot = x8/1
  Translational System/5(ydot or x10) -> ydot = x10/1
  Translational System/6(zdot or x12) -> zdot = x12/1
  Rotational System/4(x2) -> x2/1
  Rotational System/5(x4) -> x4/1
  Rotational System/6(x6) -> x6/1

== system RobustFormationControl_IntegerModel_under_Dis/Integer Leader and four followers/Leader System/Stochastic Disturbances/Dphi1 ==
  Clock : Clock
  Divide : Product  Inputs=**  RndMeth=Zero  SaturateOnIntegerOverflow=on
  Gain : Gain  Gain=0.001
  MATLAB Function : MATLAB Function  TreatAsAtomicUnit=on
  Scope : Scope
  Scope1 : Scope
  Scope2 : Scope
  Step : Step  Time=0  SampleTime=0.01
  Step1 : Step  Time=31  After=-1  SampleTime=0.01
  Sum : Sum
  Dphi1 : Outport
  wires:
  Divide/1 -> Gain/1
  Step1/1 -> Sum/2
  Sum/1 -> Scope2/1, Divide/2
  Step/1 -> Sum/1
  MATLAB Function/1(Dphi1) -> Scope/1, Divide/1
  Clock/1 -> MATLAB Function/1(t)
  Gain/1 -> Dphi1/1, Scope1/1

== system RobustFormationControl_IntegerModel_under_Dis/Integer Leader and four followers/Leader System/Stochastic Disturbances/Dphi2 ==
  Clock : Clock
  Divide : Product  Inputs=**  RndMeth=Zero  SaturateOnIntegerOverflow=on
  Gain : Gain  Gain=0.001
  MATLAB Function : MATLAB Function  TreatAsAtomicUnit=on
  Scope : Scope
  Scope1 : Scope
  Scope2 : Scope
  Step : Step  Time=0  SampleTime=0.01
  Step1 : Step  Time=31  After=-1  SampleTime=0.01
  Sum : Sum
  Dphi2 : Outport
  wires:
  Clock/1 -> MATLAB Function/1(t)
  MATLAB Function/1(Dphi2) -> Divide/1, Scope/1
  Step/1 -> Sum/1
  Sum/1 -> Divide/2, Scope2/1
  Step1/1 -> Sum/2
  Divide/1 -> Gain/1
  Gain/1 -> Scope1/1, Dphi2/1

== system RobustFormationControl_IntegerModel_under_Dis/Integer Leader and four followers/Leader System/Stochastic Disturbances/Dphi3 ==
  Clock : Clock
  Divide : Product  Inputs=**  RndMeth=Zero  SaturateOnIntegerOverflow=on
  MATLAB Function : MATLAB Function  TreatAsAtomicUnit=on
  Scope : Scope
  Scope1 : Scope
  Scope2 : Scope
  Step : Step  Time=0  SampleTime=0.01
  Step1 : Step  Time=31  After=-1  SampleTime=0.01
  Sum : Sum
  Dphi3 : Outport
  wires:
  Divide/1 -> Dphi3/1, Scope1/1
  Step1/1 -> Sum/2
  Sum/1 -> Scope2/1, Divide/2
  Step/1 -> Sum/1
  MATLAB Function/1(Dphi3) -> Scope/1, Divide/1
  Clock/1 -> MATLAB Function/1(t)

== system RobustFormationControl_IntegerModel_under_Dis/Integer Leader and four followers/Leader System/Stochastic Disturbances/Dpx ==
  Clock : Clock
  Divide : Product  Inputs=**  RndMeth=Zero  SaturateOnIntegerOverflow=on
  Gain : Gain  Gain=2
  MATLAB Function : MATLAB Function  TreatAsAtomicUnit=on
  Scope : Scope
  Scope1 : Scope
  Scope2 : Scope
  Step : Step  Time=5  SampleTime=0.01
  Step1 : Step  Time=15  After=-1  SampleTime=0.01
  Sum : Sum
  Dpx : Outport
  wires:
  Divide/1 -> Gain/1
  Step1/1 -> Sum/2
  Sum/1 -> Scope2/1, Divide/2
  Step/1 -> Sum/1
  MATLAB Function/1(Dpx) -> Scope/1, Divide/1
  Clock/1 -> MATLAB Function/1(t)
  Gain/1 -> Scope1/1, Dpx/1

== system RobustFormationControl_IntegerModel_under_Dis/Integer Leader and four followers/Leader System/Stochastic Disturbances/Dpy ==
  Clock : Clock
  Divide : Product  Inputs=**  RndMeth=Zero  SaturateOnIntegerOverflow=on
  Gain : Gain  Gain=2
  MATLAB Function : MATLAB Function  TreatAsAtomicUnit=on
  Scope : Scope
  Scope1 : Scope
  Scope2 : Scope
  Step : Step  Time=10  SampleTime=0.01
  Step1 : Step  Time=25  After=-1  SampleTime=0.01
  Sum : Sum
  Dpy : Outport
  wires:
  Divide/1 -> Gain/1
  Step1/1 -> Sum/2
  Sum/1 -> Scope2/1, Divide/2
  Step/1 -> Sum/1
  MATLAB Function/1(Dpy) -> Scope/1, Divide/1
  Clock/1 -> MATLAB Function/1(t)
  Gain/1 -> Dpy/1, Scope1/1

== system RobustFormationControl_IntegerModel_under_Dis/Integer Leader and four followers/Leader System/Stochastic Disturbances/Dpz ==
  Clock : Clock
  Divide : Product  Inputs=**  RndMeth=Zero  SaturateOnIntegerOverflow=on
  MATLAB Function : MATLAB Function  TreatAsAtomicUnit=on
  Scope : Scope
  Scope1 : Scope
  Scope2 : Scope
  Step : Step  Time=20  SampleTime=0.01
  Step1 : Step  Time=31  After=-1  SampleTime=0.01
  Sum : Sum
  Dpz : Outport
  wires:
  Divide/1 -> Dpz/1, Scope1/1
  Step1/1 -> Sum/2
  Sum/1 -> Scope2/1, Divide/2
  Step/1 -> Sum/1
  MATLAB Function/1(Dpz) -> Scope/1, Divide/1
  Clock/1 -> MATLAB Function/1(t)

== system RobustFormationControl_IntegerModel_under_Dis/Integer Leader and four followers/Leader System/Uncertainity/uncertainity in mass ==
  Constant : Constant  Value=-Ktx
  Constant1 : Constant  Value=-Kty
  Constant2 : Constant  Value=-Ktz
  Constant3 : Constant
  Constant4 : Constant
  Constant5 : Constant
  Constant6 : Constant  Commented=on  Value=m
  Divide{,1..5} (6 alike) : Product  Inputs=*/  RndMeth=Zero  SaturateOnIntegerOverflow=on
  Scope : Scope
  Stair Generator : eeStairGenerator/Stair Generator  LabelModeActiveChoice=Discrete  TimeInput=[0 8 13 19 25]  AmplitudeInput=[0.486 0.3 0.65 0.8 0.486]  SampleTime=0.001  RepeatPattern=off  OutDataTypeStr=double
      settings: LibrarySourceBlock=ee_sl_lib/General Control/Stair Generator
  Stair Generator1 : eeStairGenerator/Stair Generator  Commented=on  LabelModeActiveChoice=Discrete  TimeInput=[0 5 9 15 26]  AmplitudeInput=[0.3 0.486 0.2 0.8 0.486]  SampleTime=0.001  RepeatPattern=off  OutDataTypeStr=double
      settings: LibrarySourceBlock=ee_sl_lib/General Control/Stair Generator
  To Workspace : ToWorkspace  VariableName=Vm  SampleTime=-1
  tag scope: a4D=global, a5D=global, a6D=global, b4D=global, b5D=global, b6D=global, mV=global
  wires:
  [mV] -> Divide4/2
  Stair Generator/1 -> [mV], To Workspace/1, Scope/1
  [mV] -> Divide/2
  Constant5/1 -> Divide5/1
  Divide5/1 -> [b6D]
  Divide2/1 -> [a6D]
  [mV] -> Divide3/2
  Constant4/1 -> Divide4/1
  Divide/1 -> [a4D]
  [mV] -> Divide5/2
  [mV] -> Divide2/2
  Constant3/1 -> Divide3/1
  Divide4/1 -> [b5D]
  Constant1/1 -> Divide1/1
  Divide1/1 -> [a5D]
  Divide3/1 -> [b4D]
  Constant/1 -> Divide/1
  Constant2/1 -> Divide2/1
  [mV] -> Divide1/2

== system RobustFormationControl_IntegerModel_under_Dis/Integer Leader and four followers/Leader System/Uncertainity/uncertainity in moments of inertia ==
  Constant : Constant  Value=-Jr
  Constant1 : Constant  Commented=on  Value=Iyy
  Constant10 : Constant  Value=L
  Constant2 : Constant  Commented=on  Value=Izz
  Constant3 : Constant  Value=Jr
  Constant4 : Constant  Value=-Kfz
  Constant5 : Constant  Value=-Kfx
  Constant6 : Constant  Commented=on  Value=Ixx
  Constant7 : Constant  Value=-Kfy
  Constant8 : Constant  Value=d
  Constant9 : Constant  Value=L
  Divide{1..11} (11 alike) : Product  Inputs=*/  RndMeth=Zero  SaturateOnIntegerOverflow=on
  Gain : Gain  Gain=Ixx
  Gain1 : Gain  Gain=Iyy
  Gain2 : Gain  Gain=Izz
  Goto4 : Goto  Commented=on  GotoTag=VIxx  TagVisibility=global
  Goto5 : Goto  Commented=on  GotoTag=VIyy  TagVisibility=global
  Goto6 : Goto  Commented=on  GotoTag=VIzz  TagVisibility=global
  Scope : Scope  Commented=on
  Scope1 : Scope  Commented=on
  Scope2 : Scope  Commented=on
  Stair Generator : eeStairGenerator/Stair Generator  LabelModeActiveChoice=Discrete  TimeInput=[0 8 13 20 26]  AmplitudeInput=[1 1.5 0.8 2 1]  SampleTime=0.001  RepeatPattern=off  OutDataTypeStr=double
      settings: LibrarySourceBlock=ee_sl_lib/General Control/Stair Generator
  Stair Generator1 : eeStairGenerator/Stair Generator  LabelModeActiveChoice=Discrete  TimeInput=[0 8 13 20 26]  AmplitudeInput=[1 1.2 0.6 2 1]  SampleTime=0.001  RepeatPattern=off  OutDataTypeStr=double
      settings: LibrarySourceBlock=ee_sl_lib/General Control/Stair Generator
  Stair Generator2 : eeStairGenerator/Stair Generator  LabelModeActiveChoice=Discrete  TimeInput=[0 7 11 18 24]  AmplitudeInput=[1 1.6 0.7 2 1]  SampleTime=0.001  RepeatPattern=off  OutDataTypeStr=double
      settings: LibrarySourceBlock=ee_sl_lib/General Control/Stair Generator
  Sum : Sum  Inputs=+-
  Sum1 : Sum  Inputs=+-
  Sum2 : Sum  Inputs=+-
  To Workspace : ToWorkspace  VariableName=VIxx  SampleTime=-1
  To Workspace1 : ToWorkspace  VariableName=VIyy  SampleTime=-1
  To Workspace2 : ToWorkspace  VariableName=VIzz  SampleTime=-1
  tag scope: VIxx=global, VIyy=global, VIzz=global, a1D=global, a2D=global, a3D=global, b1D=global, b2D=global, b3D=global, c1D=global, c2D=global, c3D=global, d1D=global, d2D=global
  wires:
  [VIxx] -> Divide3/2
  Sum/1 -> Divide3/1
  Stair Generator/1 -> Gain/1
  Gain/1 -> [VIxx], To Workspace/1, Scope/1
  Gain1/1 -> To Workspace1/1, [VIyy], Scope1/1
  Stair Generator1/1 -> Gain1/1
  Stair Generator2/1 -> Gain2/1
  Gain2/1 -> To Workspace2/1, [VIzz], Scope2/1
  [VIyy] -> Sum/1
  [VIzz] -> Sum/2
  Divide3/1 -> [a1D]
  Constant2/1 -> Goto6/1
  Constant1/1 -> Goto5/1
  Constant6/1 -> Goto4/1
  Divide1/1 -> [a2D]
  [VIxx] -> Sum1/2
  [VIzz] -> Sum1/1
  Sum1/1 -> Divide1/1
  [VIyy] -> Divide1/2
  [VIzz] -> Divide2/2
  Sum2/1 -> Divide2/1
  [VIxx] -> Sum2/1
  [VIyy] -> Sum2/2
  Divide2/1 -> [a3D]
  Divide4/1 -> [b1D]
  [VIxx] -> Divide4/2
  Constant/1 -> Divide4/1
  Divide5/1 -> [b2D]
  [VIyy] -> Divide5/2
  Constant3/1 -> Divide5/1
  Divide6/1 -> [b3D]
  [VIzz] -> Divide6/2
  Constant4/1 -> Divide6/1
  Constant5/1 -> Divide7/1
  [VIxx] -> Divide7/2
  Divide7/1 -> [c1D]
  Divide8/1 -> [c2D]
  [VIyy] -> Divide8/2
  Constant7/1 -> Divide8/1
  Constant8/1 -> Divide9/1
  [VIzz] -> Divide9/2
  Divide9/1 -> [c3D]
  [VIyy] -> Divide11/2
  Constant10/1 -> Divide11/1
  Divide10/1 -> [d1D]
  Divide11/1 -> [d2D]
  [VIxx] -> Divide10/2
  Constant9/1 -> Divide10/1

== system RobustFormationControl_IntegerModel_under_Dis/Integer Leader and four followers/Follower 1 System/Follower 1 Quadrotor Model/Control Module1/Desired System ==
  Phi_d : Inport
  Theta_d : Inport  Port=2
  Psi_d : Inport  Port=3
  xd : Inport  Port=4
  yd : Inport  Port=5
  zd : Inport  Port=6
  Derivative{,1..5} (6 alike) : Derivative
  xd1 : Outport  VectorParamsAs1DForOutWhenUnconnected=off
  xd2 : Outport  Port=2  VectorParamsAs1DForOutWhenUnconnected=off
  xd3 : Outport  Port=3  VectorParamsAs1DForOutWhenUnconnected=off
  xd4 : Outport  Port=4  VectorParamsAs1DForOutWhenUnconnected=off
  xd5 : Outport  Port=5  VectorParamsAs1DForOutWhenUnconnected=off
  xd6 : Outport  Port=6  VectorParamsAs1DForOutWhenUnconnected=off
  xd7 : Outport  Port=7  VectorParamsAs1DForOutWhenUnconnected=off
  xd8 : Outport  Port=8  VectorParamsAs1DForOutWhenUnconnected=off
  xd9 : Outport  Port=9  VectorParamsAs1DForOutWhenUnconnected=off
  xd10 : Outport  Port=10  VectorParamsAs1DForOutWhenUnconnected=off
  xd11 : Outport  Port=11  VectorParamsAs1DForOutWhenUnconnected=off
  xd12 : Outport  Port=12  VectorParamsAs1DForOutWhenUnconnected=off
  wires:
  Phi_d/1 -> Derivative/1, xd1/1
  Derivative/1 -> xd2/1
  Derivative1/1 -> xd4/1
  Theta_d/1 -> Derivative1/1, xd3/1
  Psi_d/1 -> Derivative2/1, xd5/1
  Derivative2/1 -> xd6/1
  Derivative3/1 -> xd8/1
  Derivative4/1 -> xd10/1
  Derivative5/1 -> xd12/1
  xd/1 -> Derivative3/1, xd7/1
  yd/1 -> Derivative4/1, xd9/1
  zd/1 -> Derivative5/1, xd11/1

== system RobustFormationControl_IntegerModel_under_Dis/Integer Leader and four followers/Follower 1 System/Follower 1 Quadrotor Model/Control Module1/Omega Equations ==
  U1 : Inport
  U2 : Inport  Port=2
  U3 : Inport  Port=3
  U4 : Inport  Port=4
  Add1 : Sum  Inputs=+--
  Add2 : Sum  Inputs=+++
  Add3 : Sum  Inputs=++-
  Add5 : Sum  Inputs=+-+
  Control Inputs : Subsystem
  Gain11 : Gain  Gain=1/(4*b)
  Gain12 : Gain  Gain=1/(4*d)
  Gain7 : Gain  Gain=1/(2*b)
  Gain8 : Gain  Gain=1/(2*b)
  Omega : Outport  VectorParamsAs1DForOutWhenUnconnected=off
  wires:
  Add5/1 -> Control Inputs/1(w1_sqt)
  Add1/1 -> Control Inputs/2(w2_sqt)
  Add2/1 -> Control Inputs/3(w3_sqt)
  Gain11/1 -> Add5/1, Add3/1, Add2/1, Add1/1
  Gain12/1 -> Add5/3, Add2/3, Add3/3, Add1/3
  Gain7/1 -> Add5/2, Add2/2
  Gain8/1 -> Add3/2, Add1/2
  U4/1 -> Gain12/1
  U1/1 -> Gain11/1
  U3/1 -> Gain7/1
  U2/1 -> Gain8/1
  Add3/1 -> Control Inputs/4(w4_sqt)
  Control Inputs/1(Omega) -> Omega/1

== system RobustFormationControl_IntegerModel_under_Dis/Integer Leader and four followers/Follower 1 System/Follower 1 Quadrotor Model/Control Module1/Subsystem ==
  Ux : Inport
  Uy : Inport  Port=2
  Psi_d : Inport  Port=3
  Subsystem : Subsystem
  Subsystem1 : Subsystem
  Phi_d : Outport  VectorParamsAs1DForOutWhenUnconnected=off
  Theta_d : Outport  Port=2  VectorParamsAs1DForOutWhenUnconnected=off
  wires:
  Ux/1 -> Subsystem1/1(Ux), Subsystem/1(Ux)
  Uy/1 -> Subsystem1/2(Uy), Subsystem/2(Uy)
  Psi_d/1 -> Subsystem1/3(Psi_d), Subsystem/3(Psi_d)
  Subsystem/1(Phi_d) -> Subsystem1/4(Phi_d), Phi_d/1
  Subsystem1/1(Theta_d) -> Theta_d/1

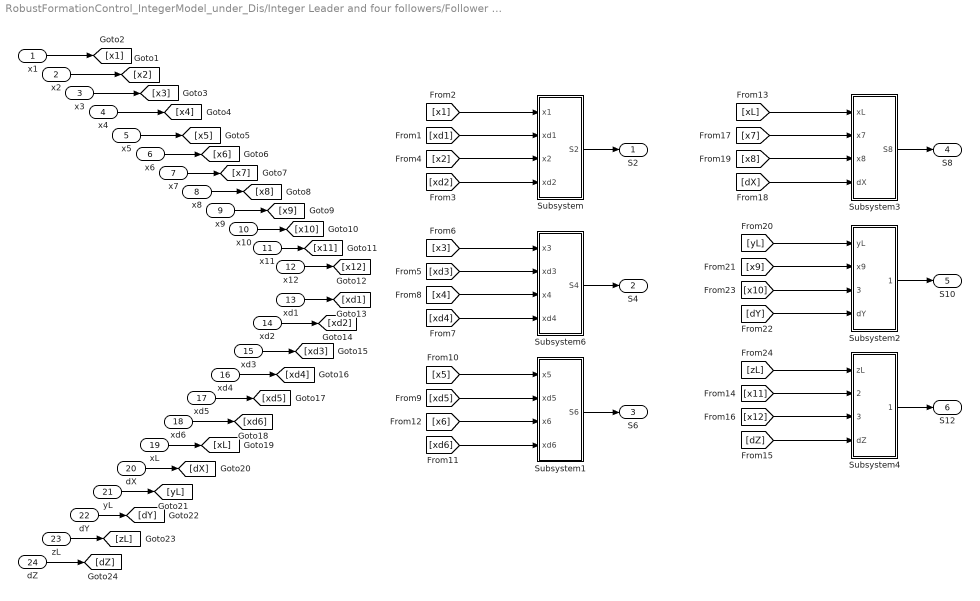
== system RobustFormationControl_IntegerModel_under_Dis/Integer Leader and four followers/Follower 1 System/Follower 1 Quadrotor Model/Control Module1/Subsystem1 ==
  x1 : Inport
  x2 : Inport  Port=2
  x3 : Inport  Port=3
  x4 : Inport  Port=4
  x5 : Inport  Port=5
  x6 : Inport  Port=6
  x7 : Inport  Port=7
  x8 : Inport  Port=8
  x9 : Inport  Port=9
  x10 : Inport  Port=10
  x11 : Inport  Port=11
  x12 : Inport  Port=12
  xd1 : Inport  Port=13
  xd2 : Inport  Port=14
  xd3 : Inport  Port=15
  xd4 : Inport  Port=16
  xd5 : Inport  Port=17
  xd6 : Inport  Port=18
  xL : Inport  Port=19
  dX : Inport  Port=20
  yL : Inport  Port=21
  dY : Inport  Port=22
  zL : Inport  Port=23
  dZ : Inport  Port=24
  Subsystem : Subsystem
  Subsystem1 : Subsystem
  Subsystem2 : Subsystem
  Subsystem3 : Subsystem
  Subsystem4 : Subsystem
  Subsystem6 : Subsystem
  S2 : Outport  VectorParamsAs1DForOutWhenUnconnected=off
  S4 : Outport  Port=2  VectorParamsAs1DForOutWhenUnconnected=off
  S6 : Outport  Port=3  VectorParamsAs1DForOutWhenUnconnected=off
  S8 : Outport  Port=4  VectorParamsAs1DForOutWhenUnconnected=off
  S10 : Outport  Port=5  VectorParamsAs1DForOutWhenUnconnected=off
  S12 : Outport  Port=6  VectorParamsAs1DForOutWhenUnconnected=off
  wires:
  x1/1 -> [x1]
  x2/1 -> [x2]
  x3/1 -> [x3]
  x4/1 -> [x4]
  x5/1 -> [x5]
  x6/1 -> [x6]
  x7/1 -> [x7]
  x8/1 -> [x8]
  x9/1 -> [x9]
  x10/1 -> [x10]
  x11/1 -> [x11]
  x12/1 -> [x12]
  xd1/1 -> [xd1]
  dY/1 -> [dY]
  xd2/1 -> [xd2]
  xd3/1 -> [xd3]
  xd4/1 -> [xd4]
  xd5/1 -> [xd5]
  xd6/1 -> [xd6]
  xL/1 -> [xL]
  dX/1 -> [dX]
  yL/1 -> [yL]
  zL/1 -> [zL]
  dZ/1 -> [dZ]
  [x1] -> Subsystem/1(x1)
  [xd1] -> Subsystem/2(xd1)
  [x2] -> Subsystem/3(x2)
  [xd2] -> Subsystem/4(xd2)
  Subsystem/1(S2) -> S2/1
  [xd4] -> Subsystem6/4(xd4)
  [x3] -> Subsystem6/1(x3)
  [x4] -> Subsystem6/3(x4)
  [xd3] -> Subsystem6/2(xd3)
  [xd6] -> Subsystem1/4(xd6)
  [x5] -> Subsystem1/1(x5)
  [x6] -> Subsystem1/3(x6)
  [xd5] -> Subsystem1/2(xd5)
  Subsystem6/1(S4) -> S4/1
  Subsystem1/1(S6) -> S6/1
  [x9] -> Subsystem2/2(x9)
  [x10] -> Subsystem2/3(x10)
  [yL] -> Subsystem2/1(yL)
  [dY] -> Subsystem2/4(dY)
  Subsystem2/1(S10) -> S10/1
  [zL] -> Subsystem4/1(zL)
  [x8] -> Subsystem3/3(x8)
  Subsystem4/1(S12) -> S12/1
  [x12] -> Subsystem4/3(x12)
  Subsystem3/1(S8) -> S8/1
  [dZ] -> Subsystem4/4(dZ)
  [x11] -> Subsystem4/2(x11)
  [x7] -> Subsystem3/2(x7)
  [dX] -> Subsystem3/4(dX)
  [xL] -> Subsystem3/1(xL)

== system RobustFormationControl_IntegerModel_under_Dis/Integer Leader and four followers/Follower 1 System/Follower 1 Quadrotor Model/Control Module1/Subsystem10 ==
  x1 : Inport
  x3 : Inport  Port=2
  x11 : Inport  Port=3
  x12 : Inport  Port=4
  zL : Inport  Port=5
  dZ : Inport  Port=6
  S12 : Inport  Port=7
  Constant1 : Constant
  Divide1 : Product  Inputs=*/
  Divide2 : Product  Inputs=**  RndMeth=Zero  SaturateOnIntegerOverflow=on
  Gain : Gain  Commented=on  Gain=b6
  Product1 : Product
  Product2 : Product
  Subsystem : Subsystem
  Subsystem1 : Subsystem
  Subsystem2 : Subsystem
  Sum2 : Sum  Inputs=+++
  Trigonometric Function1 : Trigonometry  Operator=cos
  Trigonometric Function2 : Trigonometry  Operator=cos
  U1 : Outport  VectorParamsAs1DForOutWhenUnconnected=off
  wires:
  S12/1 -> [S12]
  dZ/1 -> [dZ]
  zL/1 -> [zL]
  x3/1 -> [x3]
  Sum2/1 -> Product2/2
  Product2/1 -> U1/1
  x11/1 -> [x11]
  x12/1 -> [x12]
  x1/1 -> [x1]
  [x11] -> Subsystem/2(x11)
  [x12] -> Subsystem1/1(x12)
  [zL] -> Subsystem1/2(zL)
  [zL] -> Subsystem/1(zL)
  [dZ] -> Subsystem/4(dZ)
  [x12] -> Subsystem/3(x12)
  [S12] -> Subsystem/5(S12)
  [x11] -> Subsystem2/2(x11)
  [S12] -> Subsystem2/5(S12)
  [x12] -> Subsystem2/3(x12)
  [zL] -> Subsystem2/1(zL)
  [dZ] -> Subsystem2/4(dZ)
  Subsystem/1(D2) -> Sum2/2
  Subsystem2/1(D3) -> Sum2/3
  Subsystem1/1(D1) -> Sum2/1
  Divide1/1 -> Product2/1
  Constant1/1 -> Divide1/1
  Trigonometric Function2/1 -> Product1/2
  Trigonometric Function1/1 -> Product1/1
  Divide2/1 -> Divide1/2
  Product1/1 -> Divide2/2
  [x1] -> Trigonometric Function1/1
  [x3] -> Trigonometric Function2/1
  [b6D] -> Divide2/1
  [dZ] -> Subsystem1/3(dZ)

== system RobustFormationControl_IntegerModel_under_Dis/Integer Leader and four followers/Follower 1 System/Follower 1 Quadrotor Model/Control Module1/Subsystem2 ==
  U1 : Inport
  x9 : Inport  Port=2
  x10 : Inport  Port=3
  yL : Inport  Port=4
  dY : Inport  Port=5
  S10 : Inport  Port=6
  Constant1 : Constant
  Divide1 : Product  Inputs=*/
  Divide2 : Product  Inputs=**  RndMeth=Zero  SaturateOnIntegerOverflow=on
  Gain1 : Gain  Commented=on  Gain=b4
  Product2 : Product
  Subsystem3 : Subsystem
  Subsystem4 : Subsystem
  Subsystem5 : Subsystem
  Sum1 : Sum  Inputs=+++
  Uy : Outport  VectorParamsAs1DForOutWhenUnconnected=off
  wires:
  S10/1 -> [S10]
  dY/1 -> [dY]
  yL/1 -> [yL]
  Product2/1 -> Uy/1
  x9/1 -> [x9]
  x10/1 -> [x10]
  U1/1 -> [U1]
  Divide1/1 -> Product2/1
  Constant1/1 -> Divide1/1
  [b5D] -> Divide2/1
  [U1] -> Divide2/2
  Divide2/1 -> Divide1/2
  [dY] -> Subsystem4/3(dY)
  [dY] -> Subsystem3/4(dY)
  Subsystem4/1(D1) -> Sum1/1
  Subsystem5/1(D3) -> Sum1/3
  [yL] -> Subsystem5/1(yL)
  Subsystem3/1(D2) -> Sum1/2
  [dY] -> Subsystem5/4(dY)
  [x9] -> Subsystem3/2(x9)
  [yL] -> Subsystem3/1(yL)
  [yL] -> Subsystem4/2(yL)
  [S10] -> Subsystem3/5(S10)
  [x9] -> Subsystem5/2(x9)
  [x10] -> Subsystem5/3(x10)
  [x10] -> Subsystem4/1(x10)
  [x10] -> Subsystem3/3(x10)
  [S10] -> Subsystem5/5(S10)
  Sum1/1 -> Product2/2

== system RobustFormationControl_IntegerModel_under_Dis/Integer Leader and four followers/Follower 1 System/Follower 1 Quadrotor Model/Control Module1/Subsystem4 ==
  x1 : Inport
  x2 : Inport  Port=2
  x4 : Inport  Port=3
  x6 : Inport  Port=4
  xd1 : Inport  Port=5
  xd2 : Inport  Port=6
  S2 : Inport  Port=7
  Omega : Inport  Port=8
  Constant : Constant
  Constant3 : Constant  Value=d1
  Derivative : Derivative
  Divide : Product  Inputs=*/
  Product2 : Product
  Subsystem : Subsystem
  Subsystem1 : Subsystem
  Subsystem2 : Subsystem
  Sum2 : Sum  Inputs=+++
  U2 : Outport  VectorParamsAs1DForOutWhenUnconnected=off
  wires:
  Constant/1 -> Divide/1
  Constant3/1 -> Divide/2
  S2/1 -> [S2]
  xd2/1 -> [xd2], Derivative/1
  Derivative/1 -> [xdDot2]
  xd1/1 -> [xd1]
  x2/1 -> [x2]
  Sum2/1 -> Product2/2
  Divide/1 -> Product2/1
  Product2/1 -> U2/1
  x4/1 -> [x4]
  x6/1 -> [x6]
  x1/1 -> [x1]
  [x1] -> Subsystem/1(x1)
  [x4] -> Subsystem1/1(x4)
  [x6] -> Subsystem1/2(x6)
  [x2] -> Subsystem1/3(x2)
  Omega/1 -> Subsystem1/4(Omega)
  [xdDot2] -> Subsystem1/5(xd2)
  [xd1] -> Subsystem/2(xd1)
  [xd2] -> Subsystem/4(xd2)
  [x2] -> Subsystem/3(x2)
  [S2] -> Subsystem/5(S2)
  [xd1] -> Subsystem2/2(xd1)
  [S2] -> Subsystem2/5(S2)
  [x2] -> Subsystem2/3(x2)
  [x1] -> Subsystem2/1(x1)
  [xd2] -> Subsystem2/4(xd2)
  Subsystem1/1(D1) -> Sum2/1
  Subsystem/1(D2) -> Sum2/2
  Subsystem2/1(D3) -> Sum2/3

== system RobustFormationControl_IntegerModel_under_Dis/Integer Leader and four followers/Follower 1 System/Follower 1 Quadrotor Model/Control Module1/Subsystem5 ==
  x5 : Inport
  x2 : Inport  Port=2
  x4 : Inport  Port=3
  x6 : Inport  Port=4
  xd5 : Inport  Port=5
  xd6 : Inport  Port=6
  S6 : Inport  Port=7
  Constant : Constant
  Constant3 : Constant  Value=c3
  Derivative : Derivative
  Divide : Product  Inputs=*/
  Product2 : Product
  Subsystem : Subsystem
  Subsystem1 : Subsystem
  Subsystem2 : Subsystem
  Sum2 : Sum  Inputs=+++
  U4 : Outport  VectorParamsAs1DForOutWhenUnconnected=off
  wires:
  Constant/1 -> Divide/1
  Constant3/1 -> Divide/2
  S6/1 -> [S6]
  xd6/1 -> [xd6], Derivative/1
  Derivative/1 -> [xdDot6]
  xd5/1 -> [xd5]
  x2/1 -> [x2]
  Sum2/1 -> Product2/2
  Divide/1 -> Product2/1
  Product2/1 -> U4/1
  x4/1 -> [x4]
  x6/1 -> [x6]
  x5/1 -> [x5]
  [x5] -> Subsystem/1(x5)
  [x4] -> Subsystem1/1(x4)
  [x6] -> Subsystem1/2(x6)
  [x2] -> Subsystem1/3(x2)
  [xdDot6] -> Subsystem1/4(xd6)
  [xd5] -> Subsystem/2(xd5)
  [xd6] -> Subsystem/4(xd6)
  [x6] -> Subsystem/3(x6)
  [S6] -> Subsystem/5(S4)
  [xd5] -> Subsystem2/2(xd5)
  [S6] -> Subsystem2/5(S6)
  [x6] -> Subsystem2/3(x6)
  [x5] -> Subsystem2/1(x5)
  [xd6] -> Subsystem2/4(xd6)
  Subsystem/1(D2) -> Sum2/2
  Subsystem2/1(D3) -> Sum2/3
  Subsystem1/1(D1) -> Sum2/1

== system RobustFormationControl_IntegerModel_under_Dis/Integer Leader and four followers/Follower 1 System/Follower 1 Quadrotor Model/Control Module1/Subsystem6 ==
  U1 : Inport
  x7 : Inport  Port=2
  x8 : Inport  Port=3
  xL : Inport  Port=4
  dX : Inport  Port=5
  S8 : Inport  Port=6
  Constant1 : Constant
  Divide1 : Product  Inputs=*/
  Divide2 : Product  Inputs=**  RndMeth=Zero  SaturateOnIntegerOverflow=on
  Gain1 : Gain  Commented=on  Gain=b4
  Product2 : Product
  Subsystem3 : Subsystem
  Subsystem4 : Subsystem
  Subsystem5 : Subsystem
  Sum1 : Sum  Inputs=+++
  Ux : Outport  VectorParamsAs1DForOutWhenUnconnected=off
  wires:
  S8/1 -> [S8]
  dX/1 -> [dX]
  xL/1 -> [xL]
  Product2/1 -> Ux/1
  x7/1 -> [x7]
  x8/1 -> [x8]
  U1/1 -> [U1]
  Divide1/1 -> Product2/1
  Constant1/1 -> Divide1/1
  [b4D] -> Divide2/1
  [U1] -> Divide2/2
  Divide2/1 -> Divide1/2
  [dX] -> Subsystem4/3(dX)
  [dX] -> Subsystem3/4(dX)
  Subsystem4/1(D1) -> Sum1/1
  Subsystem5/1(D3) -> Sum1/3
  [xL] -> Subsystem5/1(xL)
  Subsystem3/1(D2) -> Sum1/2
  [dX] -> Subsystem5/4(dX)
  [x7] -> Subsystem3/2(x7)
  [xL] -> Subsystem3/1(xL)
  [xL] -> Subsystem4/2(xL)
  [S8] -> Subsystem3/5(S8)
  [x7] -> Subsystem5/2(x7)
  [x8] -> Subsystem5/3(x8)
  [x8] -> Subsystem4/1(x8)
  [x8] -> Subsystem3/3(x8)
  [S8] -> Subsystem5/5(S8)
  Sum1/1 -> Product2/2

== system RobustFormationControl_IntegerModel_under_Dis/Integer Leader and four followers/Follower 1 System/Follower 1 Quadrotor Model/Control Module1/Subsystem8 ==
  x3 : Inport
  x2 : Inport  Port=2
  x4 : Inport  Port=3
  x6 : Inport  Port=4
  xd3 : Inport  Port=5
  xd4 : Inport  Port=6
  S4 : Inport  Port=7
  Omega : Inport  Port=8
  Constant : Constant
  Constant3 : Constant  Value=d2
  Derivative : Derivative
  Divide : Product  Inputs=*/
  Product2 : Product
  Subsystem : Subsystem
  Subsystem1 : Subsystem
  Subsystem2 : Subsystem
  Sum2 : Sum  Inputs=+++
  U3 : Outport  VectorParamsAs1DForOutWhenUnconnected=off
  wires:
  Constant/1 -> Divide/1
  Constant3/1 -> Divide/2
  S4/1 -> [S4]
  xd4/1 -> [xd4], Derivative/1
  Derivative/1 -> [xdDot4]
  xd3/1 -> [xd3]
  x2/1 -> [x2]
  Sum2/1 -> Product2/2
  Divide/1 -> Product2/1
  Product2/1 -> U3/1
  x4/1 -> [x4]
  x6/1 -> [x6]
  x3/1 -> [x3]
  [x3] -> Subsystem/1(x3)
  [x4] -> Subsystem1/1(x4)
  [x6] -> Subsystem1/2(x6)
  [x2] -> Subsystem1/3(x2)
  Omega/1 -> Subsystem1/4(Omega)
  [xdDot4] -> Subsystem1/5(xd4)
  [xd3] -> Subsystem/2(xd3)
  [xd4] -> Subsystem/4(xd4)
  [x4] -> Subsystem/3(x4)
  [S4] -> Subsystem/5(S4)
  [xd3] -> Subsystem2/2(xd3)
  [S4] -> Subsystem2/5(S4)
  [x4] -> Subsystem2/3(x4)
  [x3] -> Subsystem2/1(x3)
  [xd4] -> Subsystem2/4(xd4)
  Subsystem/1(D2) -> Sum2/2
  Subsystem2/1(D3) -> Sum2/3
  Subsystem1/1(D1) -> Sum2/1
